simulink model "macroRobot_simulator"  (R2025a)
settings: Solver=FixedStepAuto  StartTime=0.0  StopTime=120  FixedStep=TsControl  MaxStep=0.00025  RelTol=1e-3
PreLoadFcn:
  | initMacroRobotSimulator;
InitFcn:
  | initMacroRobotSimulator;
values from neighbouring files (symbols this model uses):
  initState = deg2rad([-109; +67; +71; -111; -59; +20; -18])    [initMacroRobotSimulator.m]
undefined symbols (not defined in the file or in its folder): smiData, T_b_LaserGate, T_F1_Center, T_F1_Square1, T_F1_Square2, T_F1_Z1, T_F1_Z2, TsControl, X, Y, Z
libraries: sm_lib x50, nesl_utility x13, simulink x1, matrix_library x1, lib_lowLevelController x1, lib_ForwardKinematicsMacroRobot x1, lib_highLevelController x1, lib_InverseKinematicsMacroRobotVelocity x1, lib_saturateMacroRobotPosition x1
(part 1 of 2)
settings Model: Creator=muralikarnam  LastModifiedBy=gordi
settings SolverCC: InitialStep=0.00025  AlgebraicLoopSolver=TrustRegion
settings DataIOCC: ReturnWorkspaceOutputs=off
settings DebuggingCC: UnconnectedInputMsg=warning  UnconnectedOutputMsg=warning  UnconnectedLineMsg=warning  ArithmeticOperatorsInVariantConditions=warning
settings ModelReferenceCC: EnableRefExpFcnMdlSchedulingChecks=on
settings SFSimCC: SimUseLocalCustomCode=off  CustomCodeUndefinedFunction=UseInterfaceOnly
settings RTWCC: RTWUseLocalCustomCode=off  GPUComputeCapability=3.5
settings ExplorerConfigSet: InternalSimMechanicsExplorerSettings="<ExplorerConfiguration><canonicalview>default</canonicalview><AnimationSetting><BasePlaybackSpeed>1.0</BasePlaybackSpeed><PlaybackSpeedFactor>1.0</PlaybackSpeedFactor></AnimationSetting><TilePanel><TileInfo><Tiles Columns=\"2\" Count=\"4\" Rows=\"2\"><Column Weight=\"0.5\"/><Column Weight=\"0.5\"/><Row Weight=\"0.4989\"/><Row Weight=\"0.5011\"/><Tile Height=\"1\" Width=\"1\" X=\"0\" Y=\"0\"/><Tile Height=\"1\" Width=\"1\" X=\"0\" Y=\"1\"/><Tile Height=\"1\" Width=\"1\" X=\"1\" Y=\"0\"/><Tile Height=\"1\" Width=\"1\" X=\"1\" Y=\"1\"/></Tiles></TileInfo><SceneInfo><SceneViewer><BGColor><R>1</R><G>1</G><B>1</B></BGColor><Camera><DoPerspective>off</DoPerspective><Position><X>0.889681490965632871</X><Y>-0.204858956191177222</Y><Z>0.717499386736355049</Z></Position><Center><X>0.12826853071869837</X><Y>0.556554004055757279</Y><Z>-0.0439135735105794234</Z></Center><Up><X>-0.408248290463863073</X><Y>0.408248290463863073</Y><Z>0.816496580927726145</Z></Up><ViewLimDist>1</ViewLimDist><YLim>0.942103152871131888</YLim><XLim>2.08143163867977155</XLim></Camera></SceneViewer><SceneViewer><BGColor><R>1</R><G>1</G><B>1</B></BGColor><Camera><DoPerspective>off</DoPerspective><Position><X>-0.00698647458212509065</X><Y>0.230017892417154979</Y><Z>4.04703777738695258</Z></Position><Center><X>-0.00698647458212509065</X><Y>0.230017892417154979</Y><Z>2.40693099358119156</Z></Center><Up><X>0</X><Y>1</Y><Z>-0</Z></Up><ViewLimDist>1</ViewLimDist><YLim>1.03411994695663445</YLim><XLim>2.27198843364821945</XLim></Camera></SceneViewer><SceneViewer><BGColor><R>1</R><G>1</G><B>1</B></BGColor><Camera><DoPerspective>off</DoPerspective><Position><X>0.153841985146384364</X><Y>-0.651273483880472792</Y><Z>0.065143133491425087</Z></Position><Center><X>0.153841985146384364</X><Y>0.649055207581570759</Y><Z>0.065143133491425087</Z></Center><Up><X>0</X><Y>-0</Y><Z>1</Z></Up><ViewLimDist>1</ViewLimDist><YLim>0.788860071897506732</YLim><XLim>1.74286468221093993</XLim></Camera></SceneViewer><SceneViewer><BGColor><R>1</R><G>1</G><B>1</B></BGColor><Camera><DoPerspective>off</DoPerspective><Position><X>1.46260866869952211</X><Y>0.649055169227639173</Y><Z>0.0651431279093408477</Z></Position><Center><X>0.153841982815738465</X><Y>0.649055169227639173</Y><Z>0.0651431279093408477</Z></Center><Up><X>-0</X><Y>0</Y><Z>1</Z></Up><ViewLimDist>1</ViewLimDist><YLim>0.788860071897506732</YLim><XLim>1.73314610591608353</XLim></Camera></SceneViewer></SceneInfo></TilePanel><MechEditorPanel><Cameras/><GfxPanelCameraMap/><VideoCreator><PlaybackSpeedRatio>1.0</PlaybackSpeedRatio><FrameRate>30</FrameRate><VideoFormat>Motion JPEG AVI</VideoFormat><FrameSize>auto</FrameSize></VideoCreator></MechEditorPanel></ExplorerConfiguration>"

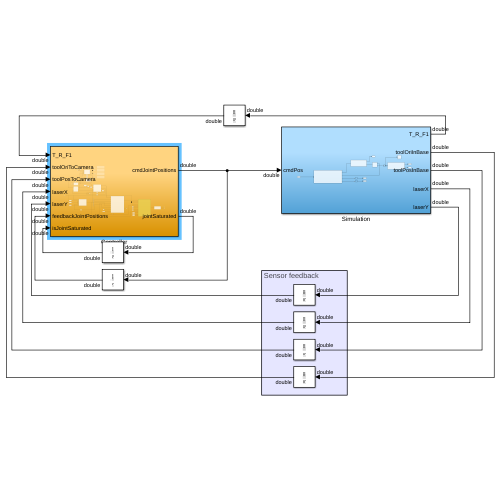
[thumbnail: Simulink's stored preview of the top-level diagram]
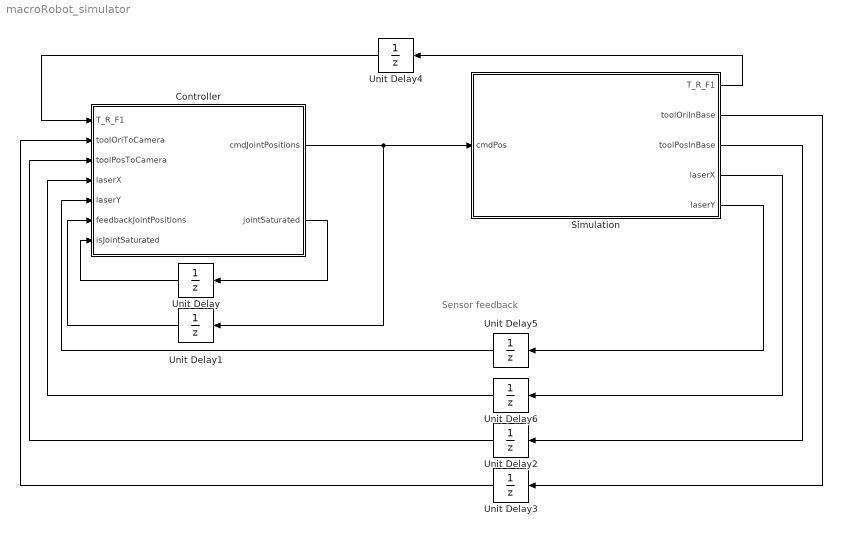
== system macroRobot_simulator ==
  note: Sensor feedback
  Controller : Subsystem
  Simulation : Subsystem
  Unit Delay : UnitDelay  SampleTime=-1  HasFrameUpgradeWarning=on
  Unit Delay1 : UnitDelay  InitialCondition=initState  SampleTime=-1  HasFrameUpgradeWarning=on
  Unit Delay{2..6} (5 alike) : UnitDelay  SampleTime=3 * TsControl  HasFrameUpgradeWarning=on
  wires:
  Controller/1(cmdJointPositions) -> Simulation/1(cmdPos), Unit Delay1/1
  Controller/2(jointSaturated) -> Unit Delay/1
  Unit Delay/1 -> Controller/7(isJointSaturated)
  Unit Delay1/1 -> Controller/6(feedbackJointPositions)
  Simulation/3(toolPosInBase) -> Unit Delay2/1
  Simulation/2(toolOriInBase) -> Unit Delay3/1
  Unit Delay2/1 -> Controller/3(toolPosToCamera)
  Unit Delay3/1 -> Controller/2(toolOriToCamera)
  Simulation/1(T_R_F1) -> Unit Delay4/1
  Unit Delay4/1 -> Controller/1(T_R_F1)
  Simulation/4(laserX) -> Unit Delay6/1
  Simulation/5(laserY) -> Unit Delay5/1
  Unit Delay6/1 -> Controller/4(laserX)
  Unit Delay5/1 -> Controller/5(laserY)

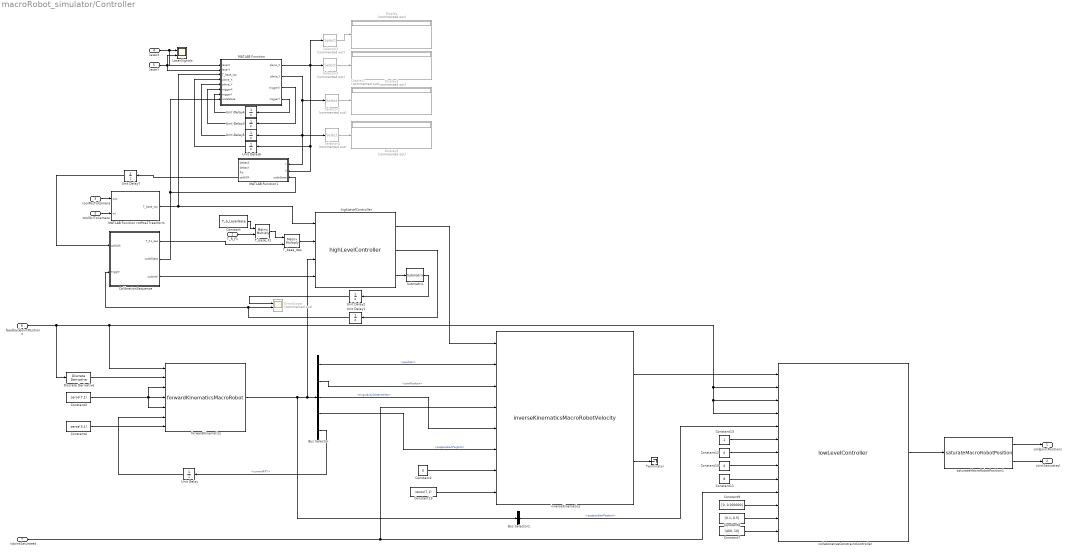
== system macroRobot_simulator/Controller ==
  T_R_F1 : Inport
  toolOriToCamera : Inport  Port=2
  toolPosToCamera : Inport  Port=3
  laserX : Inport  Port=4
  laserY : Inport  Port=5
  feedbackJointPositions : Inport  Port=6
  isJointSaturated : Inport  Port=7
  Bus Selector : BusSelector  OutputSignals=jacobian,jointPosition,singularityDistanceVec,posJacobianPerJoint,currentRPY
  Bus Selector1 : BusSelector  OutputSignals=posJacobianPerJoint
  CalibrationSequence : Stateflow chart  TreatAsAtomicUnit=on
      settings: PortSchema="{\"entries\":[{\"content\":{\"sides\":[{\"content\":{\"connectorIds\":[\"In2\",\"In1\"]},\"type\":\"ConnectorPlacement.EquallySpacedRectSide\",\"uuid\":\"ba4e8509-f946-41ef-8a94-f9774c0ab56e\"},{\"content\":{\"connectorIds\":[\"Out1\",\"Out3\",\"Out2\"],\"side\":\"RIGHT\"},\"type\":\"ConnectorPlacement.EquallySpacedRectSide\",\"uuid\":\"fc30842f-df1e-47fb-bf57-f6f1ca01699a\"},{\"content\":{\"side\":\"TOP\"},\"type\":\"ConnectorPlacement.EquallySpacedRectSide\",\"uuid\":\"47ae690f-5295-4d29-a2fc-2dde971158dc\"}]},\"type\":\"ConnectorPlacement.EquallySpacedConnector\",\"uuid\":\"3427ad9d-5ce5-4e5d-b7e5-c1727f5cb037\"}],\"packageUris\":[\"http://schema.mathworks.com/mf0/Connector/R2020b\"],\"version\":\"1.0\"}"
  Constant : Constant  Value=T_b_LaserGate
  Constant10 : Constant  Value=0  OutDataTypeStr=boolean
  Constant11 : Constant  Value=8  OutDataTypeStr=uint8
  Constant12 : Constant  Value=0  OutDataTypeStr=boolean
  Constant13 : Constant
  Constant15 : Constant  Value=zeros(7,1)
  Constant2 : Constant  Value=0
  Constant3 : Constant  Value=zeros(7,1)
  Constant4 : Constant  Value=zeros(3,1)
  Constant7 : Constant  Value=[400; 10]
  Constant8 : Constant  Value=[0.1; 0.5]
  Constant9 : Constant  Value=[0, 0.000000]
  Discrete Derivative : simulink/Discrete/Discrete Derivative  gainval=1.0  ICPrevScaledInput=0.0  OutMin=[]  OutMax=[]  OutDataType=fixdt(1, 16)  OutScaling=2^-10  DoSatur=off
  Display{,1..3} (4 alike) : Display  Commented=on
  ErrorScope : Scope  Commented=on  NumInputPorts=2
      settings: Title=ErrorPose & trigger  ActiveDisplayYMinimum=-1.2794998753501146  ActiveDisplayYMaximum=2.7547759189623635
  LaserSignals : Scope  NumInputPorts=2
      settings: Title=ErrorPose & trigger  ActiveDisplayYMinimum=-1.1952916064245291  ActiveDisplayYMaximum=2.3134323945660178  DataLoggingVariableName=ScopeData2
  MATLAB Function : MATLAB Function  TreatAsAtomicUnit=on
  MATLAB Function rotPos2Trasnform : MATLAB Function  TreatAsAtomicUnit=on
  MATLAB Function1 : MATLAB Function  TreatAsAtomicUnit=on
  Selector1 : Selector  Commented=on  NumberOfDimensions=3  InputPortWidth=3  IndexOptions=Index vector (dialog),Index vector (dialog),Index vector (dialog)  Indices=[1 2 3],[1 2],1  OutputSizes=1,1,1
  Selector2 : Selector  Commented=on  NumberOfDimensions=3  InputPortWidth=3  IndexOptions=Index vector (dialog),Index vector (dialog),Index vector (dialog)  Indices=[1 2 3],[1 2],1  OutputSizes=1,1,1
  Selector3 : Selector  Commented=on  NumberOfDimensions=3  InputPortWidth=3  IndexOptions=Index vector (dialog),Index vector (dialog),Index vector (dialog)  Indices=[1 2 3],[1 2],2  OutputSizes=1,1,1
  Selector4 : Selector  Commented=on  NumberOfDimensions=3  InputPortWidth=3  IndexOptions=Index vector (dialog),Index vector (dialog),Index vector (dialog)  Indices=[1 2 3],[1 2],2  OutputSizes=1,1,1
  Submatrix : matrix_library/Submatrix  RowSpan=Range of rows  RowStartMode=First  RowStartIndex=1  RowEndMode=Index  RowEndIndex=3  ColSpan=All columns  ColStartMode=First  ColStartIndex=1  ColEndMode=Last  ColEndIndex=1
  T_base_F1 : Product  Multiplication=Matrix(*)
  T_base_des : Product  Multiplication=Matrix(*)
  Terminator : Terminator
  Unit Delay{,1..4,7} (6 alike) : UnitDelay  SampleTime=-1  HasFrameUpgradeWarning=on
  Unit Delay5 : UnitDelay  InitialCondition=zeros(3,2,2,3)  SampleTime=-1  HasFrameUpgradeWarning=on
  Unit Delay6 : UnitDelay  InitialCondition=zeros(3,2,2,3)  SampleTime=-1  HasFrameUpgradeWarning=on
  collaborativeConstraintController : lib_lowLevelController/lowLevelController  SystemSampleTime=-1  VariantActivationTime=update diagram  EmptyChoice=off  PassThrough=off  PassThroughVariantControl=(default)  EmptyChoiceVariantControl=(default)  AllowFlexibleInterface=on  Latency=0  AutoFrameSizeCalculation=off
  forwardKinematics : lib_ForwardKinematicsMacroRobot/forwardKinematicsMacroRobot  SystemSampleTime=-1  VariantActivationTime=update diagram  EmptyChoice=off  PassThrough=off  PassThroughVariantControl=(default)  EmptyChoiceVariantControl=(default)  AllowFlexibleInterface=on  Latency=0  AutoFrameSizeCalculation=off
  highLevelController : lib_highLevelController/highLevelController  SystemSampleTime=-1  VariantActivationTime=update diagram  EmptyChoice=off  PassThrough=off  PassThroughVariantControl=(default)  EmptyChoiceVariantControl=(default)  AllowFlexibleInterface=on  Latency=0  AutoFrameSizeCalculation=off
  inverseKinematics : lib_InverseKinematicsMacroRobotVelocity/inverseKinematicsMacroRobotVelocity  SystemSampleTime=-1  VariantActivationTime=update diagram  EmptyChoice=off  PassThrough=off  PassThroughVariantControl=(default)  EmptyChoiceVariantControl=(default)  AllowFlexibleInterface=on  Latency=0  AutoFrameSizeCalculation=off
  saturateMacroRobotPosition1 : lib_saturateMacroRobotPosition/saturateMacroRobotPosition  SystemSampleTime=-1  VariantActivationTime=update diagram  EmptyChoice=off  PassThrough=off  PassThroughVariantControl=(default)  EmptyChoiceVariantControl=(default)  AllowFlexibleInterface=on  Latency=0  AutoFrameSizeCalculation=off
  cmdJointPositions : Outport  VectorParamsAs1DForOutWhenUnconnected=off
  jointSaturated : Outport  Port=2  VectorParamsAs1DForOutWhenUnconnected=off
  wires:
  feedbackJointPositions/1 -> Discrete Derivative/1, collaborativeConstraintController/2, collaborativeConstraintController/3, collaborativeConstraintController/4, forwardKinematics/1
  Unit Delay/1 -> forwardKinematics/6
  Bus Selector/1 -> inverseKinematics/2  "<jacobian>"
  Constant8/1 -> collaborativeConstraintController/12
  Constant2/1 -> inverseKinematics/7
  inverseKinematics/1 -> collaborativeConstraintController/1
  Constant7/1 -> collaborativeConstraintController/13
  Constant3/1 -> forwardKinematics/3, forwardKinematics/5, forwardKinematics/4
  Bus Selector/2 -> inverseKinematics/3  "<jointPosition>"
  Bus Selector/5 -> Unit Delay/1  "<currentRPY>"
  Constant9/1 -> collaborativeConstraintController/11
  Discrete Derivative/1 -> forwardKinematics/2
  Constant12/1 -> collaborativeConstraintController/7
  Constant4/1 -> forwardKinematics/7
  forwardKinematics/1 -> highLevelController/3, Bus Selector/1, Bus Selector1/1
  Constant11/1 -> collaborativeConstraintController/9
  Constant10/1 -> collaborativeConstraintController/8
  Constant13/1 -> collaborativeConstraintController/6
  Bus Selector1/1 -> collaborativeConstraintController/5  "<posJacobianPerJoint>"
  Bus Selector/4 -> inverseKinematics/6  "<posJacobianPerJoint>"
  inverseKinematics/2 -> Terminator/1
  Bus Selector/3 -> inverseKinematics/5  "<singularityDistanceVec>"
  isJointSaturated/1 -> inverseKinematics/4, collaborativeConstraintController/10
  Constant15/1 -> inverseKinematics/8
  saturateMacroRobotPosition1/1 -> cmdJointPositions/1
  collaborativeConstraintController/1 -> saturateMacroRobotPosition1/1
  saturateMacroRobotPosition1/2 -> jointSaturated/1
  highLevelController/1 -> inverseKinematics/1
  toolOriToCamera/1 -> MATLAB Function rotPos2Trasnform/2(ori)
  toolPosToCamera/1 -> MATLAB Function rotPos2Trasnform/1(pos)
  MATLAB Function rotPos2Trasnform/1(T_base_tcp) -> highLevelController/1, MATLAB Function/3(T_base_tcp)
  highLevelController/2 -> Unit Delay1/1
  Unit Delay1/1 -> CalibrationSequence/1(trigger), ErrorScope/2
  Constant/1 -> T_base_F1/1
  T_base_F1/1 -> T_base_des/1
  T_R_F1/1 -> T_base_F1/2
  T_base_des/1 -> highLevelController/2
  CalibrationSequence/1(T_F1_des) -> T_base_des/2
  highLevelController/3 -> Submatrix/1
  Unit Delay2/1 -> ErrorScope/1
  Submatrix/1 -> Unit Delay2/1
  CalibrationSequence/2(codeVel) -> highLevelController/4
  laserY/1 -> MATLAB Function/2(laserY), LaserSignals/2
  laserX/1 -> MATLAB Function/1(laserX), LaserSignals/1
  MATLAB Function/4(triggerY) -> Unit Delay4/1
  Unit Delay3/1 -> MATLAB Function/6("triggerX ")
  Unit Delay4/1 -> MATLAB Function/7("triggerY ")
  MATLAB Function/1(plane_X) -> Selector2/1, Selector3/1, MATLAB Function1/2(X), Unit Delay6/1
  MATLAB Function/2(plane_Y) -> MATLAB Function1/1(Y), Unit Delay5/1, Selector4/1, Selector1/1
  MATLAB Function/3(triggerX) -> Unit Delay3/1
  Selector2/1 -> Display/1
  Selector1/1 -> Display1/1
  CalibrationSequence/3(codeState) -> MATLAB Function/8(codeState), MATLAB Function1/3(codeState)
  Selector3/1 -> Display2/1
  Selector4/1 -> Display3/1
  Unit Delay5/1 -> MATLAB Function/5("plane_Y ")
  Unit Delay6/1 -> MATLAB Function/4("plane_X ")
  MATLAB Function1/4(calibOK) -> Unit Delay7/1
  Unit Delay7/1 -> CalibrationSequence/2(calibOK)

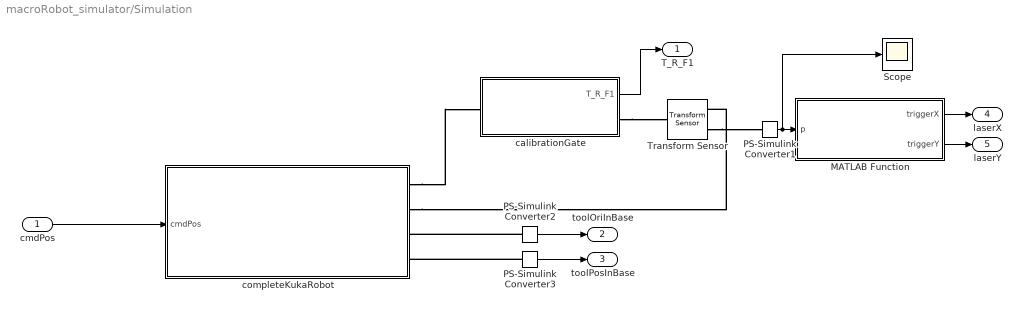
== system macroRobot_simulator/Simulation ==
  cmdPos : Inport
  MATLAB Function : MATLAB Function  TreatAsAtomicUnit=on
  PS-Simulink Converter1 : nesl_utility/PS-Simulink Converter  PhysicalDomain=network_engine_domain  SubClassName=ps_output  LeftPortType=input  RightPortType=output  PseudoPeriodic=off  Frequencies=[]  VectorFormat=inherit  Unit=inherit  AffineConversion=off
  PS-Simulink Converter2 : nesl_utility/PS-Simulink Converter  PhysicalDomain=network_engine_domain  SubClassName=ps_output  LeftPortType=input  RightPortType=output  PseudoPeriodic=off  Frequencies=[]  VectorFormat=inherit  Unit=inherit  AffineConversion=off
  PS-Simulink Converter3 : nesl_utility/PS-Simulink Converter  PhysicalDomain=network_engine_domain  SubClassName=ps_output  LeftPortType=input  RightPortType=output  PseudoPeriodic=off  Frequencies=[]  VectorFormat=inherit  Unit=inherit  AffineConversion=off
  Scope : Scope
  Transform Sensor : sm_lib/Frames and Transforms/Transform Sensor  MeasurementFrame=World  RotationSequence=XYX  SenseAngle=off  SenseAxis=off  SenseQ=off  SenseR=off  SenseRotationSequence=off  SenseOmegaX=off  SenseOmegaY=off  SenseOmegaZ=off  SenseOmega=off  SenseQDot=off  SenseRDot=off  SenseRotationSequenceDot=off  SenseAlphaX=off  SenseAlphaY=off  SenseAlphaZ=off  SenseAlpha=off  SenseQDDot=off  SenseRDDot=off  SenseX=off  SenseY=off  SenseZ=off  SenseXYZ=on  SenseRad=off  SenseAzim=off  SenseDist=off  SenseInc=off  SenseXDot=off  SenseYDot=off  SenseZDot=off  SenseXYZDot=off  SenseRadDot=off  SenseAzimDot=off  SenseDistDot=off  SenseIncDot=off  SenseXDDot=off  SenseYDDot=off  SenseZDDot=off  SenseXYZDDot=off  SenseRadDDot=off  SenseAzimDDot=off  SenseDistDDot=off  SenseIncDDot=off
  calibrationGate : Subsystem
  completeKukaRobot : Subsystem
  T_R_F1 : Outport
  toolOriInBase : Outport  Port=2
  toolPosInBase : Outport  Port=3
  laserX : Outport  Port=4
  laserY : Outport  Port=5
  wires:
  cmdPos/1 -> completeKukaRobot/1(cmdPos)
  PS-Simulink Converter3/1 -> toolPosInBase/1
  PS-Simulink Converter2/1 -> toolOriInBase/1
  calibrationGate/1(T_R_F1) -> T_R_F1/1
  PS-Simulink Converter1/1 -> Scope/1, MATLAB Function/1(p)
  MATLAB Function/1(triggerX) -> laserX/1
  MATLAB Function/2(triggerY) -> laserY/1
  connections:
  PS-Simulink Converter3/LConn1 -- completeKukaRobot/RConn4
  PS-Simulink Converter2/LConn1 -- completeKukaRobot/RConn3
  completeKukaRobot/RConn1 -- calibrationGate/LConn1
  completeKukaRobot/RConn2 -- Transform Sensor/RConn1
  calibrationGate/RConn1 -- Transform Sensor/LConn1
  Transform Sensor/RConn2 -- PS-Simulink Converter1/LConn1

== system macroRobot_simulator/Simulation/calibrationGate ==
  laserGate : Subsystem
  tableFrame : PMIOPort  Side=Left
  LaserGate_F1 : PMIOPort  Port=2  Side=Right
  T_R_F1 : Outport
  wires:
  laserGate/1(T_R_F1) -> T_R_F1/1
  connections:
  laserGate/LConn1 -- tableFrame/RConn1
  LaserGate_F1/RConn1 -- laserGate/RConn1

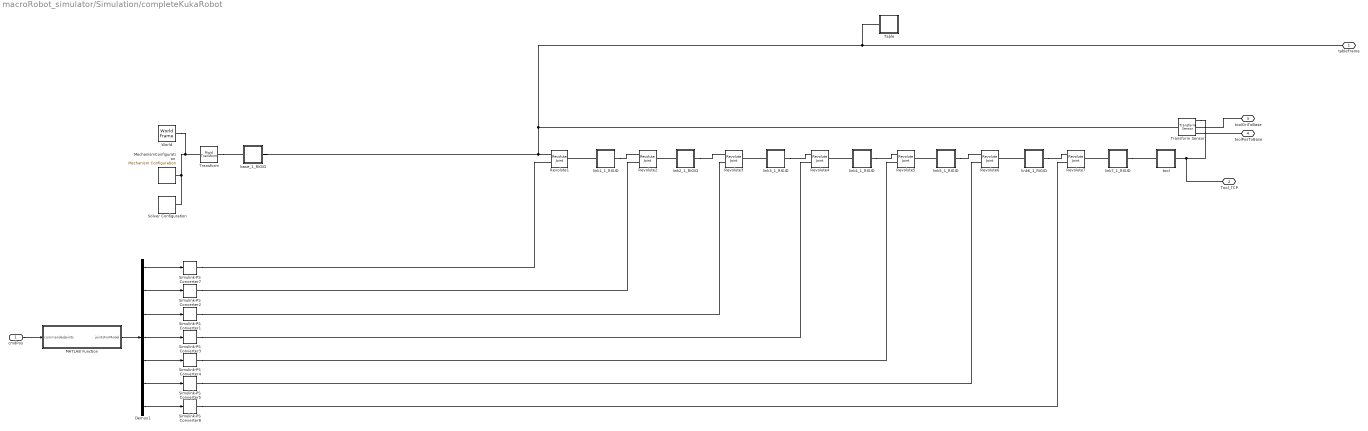
== system macroRobot_simulator/Simulation/completeKukaRobot ==
  cmdPos : Inport  PortDimensions=[7 1]
  Demux1 : Demux  Outputs=7
  MATLAB Function : MATLAB Function  TreatAsAtomicUnit=on
  MechanismConfiguration : sm_lib/Utilities/Mechanism Configuration  UniformGravity=Constant  GravityVector=[0 -9.80665 0]  GravityVectorUnits=m/s^2  LinearizationDelta=0.001  JointModeTransitionNonlinearIterations=2
  Revolute1 : sm_lib/Joints/Revolute Joint  JointMode=Normal  CompositeWrenchDir=FollowerOnBase  CompositeWrenchFrame=BaseFrame  SenseConstraintForce=off  SenseConstraintTorque=off  SenseTotalForce=off  SenseTotalTorque=off  PositionTargetSpecify=on  PositionTargetPriority=Low  PositionTargetValue=initState(1)  PositionTargetValueUnits=rad  VelocityTargetSpecify=off  VelocityTargetPriority=High  VelocityTargetValue=0  VelocityTargetValueUnits=deg/s  EquilibriumPosition=0  EquilibriumPositionUnits=rad  SpringStiffness=0  SpringStiffnessUnits=N*m/rad  DampingCoefficient=0  DampingCoefficientUnits=N*m/(rad/s)  LowerLimitSpecify=off  LowerLimitBound=-90  LowerLimitBoundUnits=deg  LowerLimitStiffness=1e4  LowerLimitStiffnessUnits=N*m/deg  LowerLimitDamping=10  LowerLimitDampingUnits=N*m/(deg/s)  LowerLimitTransitionRegionWidth=0.1  LowerLimitTransitionRegionWidthUnits=deg  UpperLimitSpecify=off  UpperLimitBound=90  UpperLimitBoundUnits=deg  UpperLimitStiffness=1e4  UpperLimitStiffnessUnits=N*m/deg  UpperLimitDamping=10  UpperLimitDampingUnits=N*m/(deg/s)  UpperLimitTransitionRegionWidth=0.1  UpperLimitTransitionRegionWidthUnits=deg  TorqueActuationMode=ComputedTorque  MotionActuationMode=InputMotion  SensePosition=off  SenseVelocity=off  SenseAcceleration=off  SenseTorqueForce=off  SenseLowerLimitTorqueForce=off  SenseUpperLimitTorqueForce=off
  Revolute2 : sm_lib/Joints/Revolute Joint  JointMode=Normal  CompositeWrenchDir=FollowerOnBase  CompositeWrenchFrame=BaseFrame  SenseConstraintForce=off  SenseConstraintTorque=off  SenseTotalForce=off  SenseTotalTorque=off  PositionTargetSpecify=on  PositionTargetPriority=Low  PositionTargetValue=initState(2)  PositionTargetValueUnits=rad  VelocityTargetSpecify=off  VelocityTargetPriority=High  VelocityTargetValue=0  VelocityTargetValueUnits=deg/s  EquilibriumPosition=0  EquilibriumPositionUnits=rad  SpringStiffness=0  SpringStiffnessUnits=N*m/rad  DampingCoefficient=0  DampingCoefficientUnits=N*m/(rad/s)  LowerLimitSpecify=off  LowerLimitBound=-90  LowerLimitBoundUnits=deg  LowerLimitStiffness=1e4  LowerLimitStiffnessUnits=N*m/deg  LowerLimitDamping=10  LowerLimitDampingUnits=N*m/(deg/s)  LowerLimitTransitionRegionWidth=0.1  LowerLimitTransitionRegionWidthUnits=deg  UpperLimitSpecify=off  UpperLimitBound=90  UpperLimitBoundUnits=deg  UpperLimitStiffness=1e4  UpperLimitStiffnessUnits=N*m/deg  UpperLimitDamping=10  UpperLimitDampingUnits=N*m/(deg/s)  UpperLimitTransitionRegionWidth=0.1  UpperLimitTransitionRegionWidthUnits=deg  TorqueActuationMode=ComputedTorque  MotionActuationMode=InputMotion  SensePosition=off  SenseVelocity=off  SenseAcceleration=off  SenseTorqueForce=off  SenseLowerLimitTorqueForce=off  SenseUpperLimitTorqueForce=off
  Revolute3 : sm_lib/Joints/Revolute Joint  JointMode=Normal  CompositeWrenchDir=FollowerOnBase  CompositeWrenchFrame=BaseFrame  SenseConstraintForce=off  SenseConstraintTorque=off  SenseTotalForce=off  SenseTotalTorque=off  PositionTargetSpecify=on  PositionTargetPriority=Low  PositionTargetValue=initState(3)  PositionTargetValueUnits=rad  VelocityTargetSpecify=off  VelocityTargetPriority=High  VelocityTargetValue=0  VelocityTargetValueUnits=deg/s  EquilibriumPosition=0  EquilibriumPositionUnits=rad  SpringStiffness=0  SpringStiffnessUnits=N*m/rad  DampingCoefficient=0  DampingCoefficientUnits=N*m/(rad/s)  LowerLimitSpecify=off  LowerLimitBound=-90  LowerLimitBoundUnits=deg  LowerLimitStiffness=1e4  LowerLimitStiffnessUnits=N*m/deg  LowerLimitDamping=10  LowerLimitDampingUnits=N*m/(deg/s)  LowerLimitTransitionRegionWidth=0.1  LowerLimitTransitionRegionWidthUnits=deg  UpperLimitSpecify=off  UpperLimitBound=90  UpperLimitBoundUnits=deg  UpperLimitStiffness=1e4  UpperLimitStiffnessUnits=N*m/deg  UpperLimitDamping=10  UpperLimitDampingUnits=N*m/(deg/s)  UpperLimitTransitionRegionWidth=0.1  UpperLimitTransitionRegionWidthUnits=deg  TorqueActuationMode=ComputedTorque  MotionActuationMode=InputMotion  SensePosition=off  SenseVelocity=off  SenseAcceleration=off  SenseTorqueForce=off  SenseLowerLimitTorqueForce=off  SenseUpperLimitTorqueForce=off
  Revolute4 : sm_lib/Joints/Revolute Joint  JointMode=Normal  CompositeWrenchDir=FollowerOnBase  CompositeWrenchFrame=BaseFrame  SenseConstraintForce=off  SenseConstraintTorque=off  SenseTotalForce=off  SenseTotalTorque=off  PositionTargetSpecify=on  PositionTargetPriority=Low  PositionTargetValue=-initState(4)  PositionTargetValueUnits=rad  VelocityTargetSpecify=off  VelocityTargetPriority=High  VelocityTargetValue=0  VelocityTargetValueUnits=deg/s  EquilibriumPosition=0  EquilibriumPositionUnits=rad  SpringStiffness=0  SpringStiffnessUnits=N*m/rad  DampingCoefficient=0  DampingCoefficientUnits=N*m/(rad/s)  LowerLimitSpecify=off  LowerLimitBound=-90  LowerLimitBoundUnits=deg  LowerLimitStiffness=1e4  LowerLimitStiffnessUnits=N*m/deg  LowerLimitDamping=10  LowerLimitDampingUnits=N*m/(deg/s)  LowerLimitTransitionRegionWidth=0.1  LowerLimitTransitionRegionWidthUnits=deg  UpperLimitSpecify=off  UpperLimitBound=90  UpperLimitBoundUnits=deg  UpperLimitStiffness=1e4  UpperLimitStiffnessUnits=N*m/deg  UpperLimitDamping=10  UpperLimitDampingUnits=N*m/(deg/s)  UpperLimitTransitionRegionWidth=0.1  UpperLimitTransitionRegionWidthUnits=deg  TorqueActuationMode=ComputedTorque  MotionActuationMode=InputMotion  SensePosition=off  SenseVelocity=off  SenseAcceleration=off  SenseTorqueForce=off  SenseLowerLimitTorqueForce=off  SenseUpperLimitTorqueForce=off
  Revolute5 : sm_lib/Joints/Revolute Joint  JointMode=Normal  CompositeWrenchDir=FollowerOnBase  CompositeWrenchFrame=BaseFrame  SenseConstraintForce=off  SenseConstraintTorque=off  SenseTotalForce=off  SenseTotalTorque=off  PositionTargetSpecify=on  PositionTargetPriority=Low  PositionTargetValue=initState(5)  PositionTargetValueUnits=rad  VelocityTargetSpecify=off  VelocityTargetPriority=High  VelocityTargetValue=0  VelocityTargetValueUnits=deg/s  EquilibriumPosition=0  EquilibriumPositionUnits=rad  SpringStiffness=0  SpringStiffnessUnits=N*m/rad  DampingCoefficient=0  DampingCoefficientUnits=N*m/(rad/s)  LowerLimitSpecify=off  LowerLimitBound=-90  LowerLimitBoundUnits=deg  LowerLimitStiffness=1e4  LowerLimitStiffnessUnits=N*m/deg  LowerLimitDamping=10  LowerLimitDampingUnits=N*m/(deg/s)  LowerLimitTransitionRegionWidth=0.1  LowerLimitTransitionRegionWidthUnits=deg  UpperLimitSpecify=off  UpperLimitBound=90  UpperLimitBoundUnits=deg  UpperLimitStiffness=1e4  UpperLimitStiffnessUnits=N*m/deg  UpperLimitDamping=10  UpperLimitDampingUnits=N*m/(deg/s)  UpperLimitTransitionRegionWidth=0.1  UpperLimitTransitionRegionWidthUnits=deg  TorqueActuationMode=ComputedTorque  MotionActuationMode=InputMotion  SensePosition=off  SenseVelocity=off  SenseAcceleration=off  SenseTorqueForce=off  SenseLowerLimitTorqueForce=off  SenseUpperLimitTorqueForce=off
  Revolute6 : sm_lib/Joints/Revolute Joint  JointMode=Normal  CompositeWrenchDir=FollowerOnBase  CompositeWrenchFrame=BaseFrame  SenseConstraintForce=off  SenseConstraintTorque=off  SenseTotalForce=off  SenseTotalTorque=off  PositionTargetSpecify=on  PositionTargetPriority=Low  PositionTargetValue=initState(6)  PositionTargetValueUnits=rad  VelocityTargetSpecify=off  VelocityTargetPriority=High  VelocityTargetValue=0  VelocityTargetValueUnits=deg/s  EquilibriumPosition=0  EquilibriumPositionUnits=rad  SpringStiffness=0  SpringStiffnessUnits=N*m/rad  DampingCoefficient=0  DampingCoefficientUnits=N*m/(rad/s)  LowerLimitSpecify=off  LowerLimitBound=-90  LowerLimitBoundUnits=deg  LowerLimitStiffness=1e4  LowerLimitStiffnessUnits=N*m/deg  LowerLimitDamping=10  LowerLimitDampingUnits=N*m/(deg/s)  LowerLimitTransitionRegionWidth=0.1  LowerLimitTransitionRegionWidthUnits=deg  UpperLimitSpecify=off  UpperLimitBound=90  UpperLimitBoundUnits=deg  UpperLimitStiffness=1e4  UpperLimitStiffnessUnits=N*m/deg  UpperLimitDamping=10  UpperLimitDampingUnits=N*m/(deg/s)  UpperLimitTransitionRegionWidth=0.1  UpperLimitTransitionRegionWidthUnits=deg  TorqueActuationMode=ComputedTorque  MotionActuationMode=InputMotion  SensePosition=off  SenseVelocity=off  SenseAcceleration=off  SenseTorqueForce=off  SenseLowerLimitTorqueForce=off  SenseUpperLimitTorqueForce=off
  Revolute7 : sm_lib/Joints/Revolute Joint  JointMode=Normal  CompositeWrenchDir=FollowerOnBase  CompositeWrenchFrame=BaseFrame  SenseConstraintForce=off  SenseConstraintTorque=off  SenseTotalForce=off  SenseTotalTorque=off  PositionTargetSpecify=on  PositionTargetPriority=Low  PositionTargetValue=initState(7)  PositionTargetValueUnits=rad  VelocityTargetSpecify=off  VelocityTargetPriority=High  VelocityTargetValue=0  VelocityTargetValueUnits=deg/s  EquilibriumPosition=0  EquilibriumPositionUnits=rad  SpringStiffness=0  SpringStiffnessUnits=N*m/rad  DampingCoefficient=0  DampingCoefficientUnits=N*m/(rad/s)  LowerLimitSpecify=off  LowerLimitBound=-90  LowerLimitBoundUnits=deg  LowerLimitStiffness=1e4  LowerLimitStiffnessUnits=N*m/deg  LowerLimitDamping=10  LowerLimitDampingUnits=N*m/(deg/s)  LowerLimitTransitionRegionWidth=0.1  LowerLimitTransitionRegionWidthUnits=deg  UpperLimitSpecify=off  UpperLimitBound=90  UpperLimitBoundUnits=deg  UpperLimitStiffness=1e4  UpperLimitStiffnessUnits=N*m/deg  UpperLimitDamping=10  UpperLimitDampingUnits=N*m/(deg/s)  UpperLimitTransitionRegionWidth=0.1  UpperLimitTransitionRegionWidthUnits=deg  TorqueActuationMode=ComputedTorque  MotionActuationMode=InputMotion  SensePosition=off  SenseVelocity=off  SenseAcceleration=off  SenseTorqueForce=off  SenseLowerLimitTorqueForce=off  SenseUpperLimitTorqueForce=off
  Simulink-PS Converter{1..5,7..8} (7 alike) : nesl_utility/Simulink-PS Converter  PhysicalDomain=network_engine_domain  SubClassName=ps_input  LeftPortType=input  RightPortType=output  PseudoPeriodic=off  Frequencies=[]  NoiseDistribution=none  NoiseParameters=[]  Unit=1  AffineConversion=off  FilteringAndDerivatives=filter  SimscapeFilterOrder=2  InputFilterTimeConstant=0.001  UdotUserProvided=0
  Solver Configuration : nesl_utility/Solver Configuration  PhysicalDomain=network_engine_domain  SubClassName=solver  LeftPortType=input  RightPortType=generic  Tones=[]  Harmonics=[]  SimulateNoise=off  Profile=off  UseLocalSampling=off  EnableSwitchedLinearOptims=on  FrequencyDomain=off  UseCCode=off  RelTol=0.001  AbsTol=0.001  MinStep=1e-09  ToWorkspace=off  RevertToSquareIcSolve=off  NumHomotopyIterations=100  PhasorMode=off  PhasorModeNumHarmonics=1  ConsistencySolver=NEWTON_XTOL_AFTER_FTOL  IndexReductionMethod=DerivativeReplacement  DoDC=off  ResidualTolerance=1e-09  ConsistencyTolSource=GLOBAL  ConsistencyAbsTol=0.001  ConsistencyRelTol=0.001  ConsistencyTolFactor=0.001  UseLocalSolver=off  LocalSolverChoice=NE_BACKWARD_EULER_ADVANCER  ResolveIndetEquations=on  FunctionEvalNumThread=1  LocalSolverSampleTime=0.001  DoFixedCost=off  MaxNonlinIter=3  MaxModeIter=2  ComputeImpulses=off  ImpulseIterations=2  LinearAlgebra=auto  LinearAlgebraNumThread=0  EquationFormulation=NE_TIME_EF  DelaysMemoryBudget=1024  AutomaticFiltering=on  FilteringTimeConstant=0.001  PartitionStorageMethod=AS_NEEDED  PartitionMemoryBudget=1024  PartitionMethod=ROBUST  MultibodyUseLocalSolver=off  MultibodyLocalSolverChoice=ODE1  MultibodyLocalSolverSampleTime=0.001
  Table : Subsystem
  Transform : sm_lib/Frames and Transforms/Rigid Transform  RotationMethod=ArbitraryAxis  FollAlignAxisA=+X  BaseAlignAxisA=+Y  FollAlignAxisB=+Y  BaseAlignAxisB=+Z  RotationStandardAxis=+Z  RotationAngle=smiData.RigidTransform(15).angle  RotationAngleUnits=rad  RotationArbitraryAxis=smiData.RigidTransform(15).axis  RotationSequenceAxes=FollowerAxes  RotationSequence=XYX  RotationSequenceAngles=[0 0 0]  RotationSequenceAnglesUnits=deg  RotationMatrix=[1 0 0; 0 1 0; 0 0 1]  Quaternion=[1 0 0 0]  TranslationMethod=Cartesian  TranslationCartesianOffset=smiData.RigidTransform(15).translation  TranslationCartesianOffsetUnits=mm  TranslationStandardAxis=+Z  TranslationStandardOffset=0  TranslationStandardOffsetUnits=m  TranslationROffset=0  TranslationROffsetUnits=m  TranslationThetaOffset=0  TranslationThetaOffsetUnits=deg  TranslationZOffset=0  TranslationZOffsetUnits=m
  Transform Sensor : sm_lib/Frames and Transforms/Transform Sensor  MeasurementFrame=Base  RotationSequence=XYX  SenseAngle=off  SenseAxis=off  SenseQ=off  SenseR=on  SenseRotationSequence=off  SenseOmegaX=off  SenseOmegaY=off  SenseOmegaZ=off  SenseOmega=off  SenseQDot=off  SenseRDot=off  SenseRotationSequenceDot=off  SenseAlphaX=off  SenseAlphaY=off  SenseAlphaZ=off  SenseAlpha=off  SenseQDDot=off  SenseRDDot=off  SenseX=off  SenseY=off  SenseZ=off  SenseXYZ=on  SenseRad=off  SenseAzim=off  SenseDist=off  SenseInc=off  SenseXDot=off  SenseYDot=off  SenseZDot=off  SenseXYZDot=off  SenseRadDot=off  SenseAzimDot=off  SenseDistDot=off  SenseIncDot=off  SenseXDDot=off  SenseYDDot=off  SenseZDDot=off  SenseXYZDDot=off  SenseRadDDot=off  SenseAzimDDot=off  SenseDistDDot=off  SenseIncDDot=off
  World : sm_lib/Frames and Transforms/World Frame
  base_1_RIGID : Subsystem
  link1_1_RIGID : Subsystem
  link2_1_RIGID : Subsystem
  link3_1_RIGID : Subsystem
  link4_1_RIGID : Subsystem
  link5_1_RIGID : Subsystem
  link6_1_RIGID : Subsystem
  link7_1_RIGID : Subsystem
  tool : Subsystem
  tableFrame : PMIOPort  Side=Right
  Tool_TCP : PMIOPort  Port=2  Side=Right
  toolOriToBase : PMIOPort  Port=3  Side=Right
  toolPosToBase : PMIOPort  Port=4  Side=Right
  wires:
  cmdPos/1 -> MATLAB Function/1(commandedJoints)
  Demux1/7 -> Simulink-PS Converter8/1
  Demux1/6 -> Simulink-PS Converter5/1
  Demux1/5 -> Simulink-PS Converter4/1
  Demux1/4 -> Simulink-PS Converter3/1
  Demux1/3 -> Simulink-PS Converter1/1
  Demux1/2 -> Simulink-PS Converter2/1
  Demux1/1 -> Simulink-PS Converter7/1
  MATLAB Function/1(jointsForModel) -> Demux1/1
  connections:
  Simulink-PS Converter2/RConn1 -- Revolute2/LConn2
  Simulink-PS Converter3/RConn1 -- Revolute4/LConn2
  Simulink-PS Converter5/RConn1 -- Revolute6/LConn2
  Simulink-PS Converter1/RConn1 -- Revolute3/LConn2
  Simulink-PS Converter4/RConn1 -- Revolute5/LConn2
  Simulink-PS Converter8/RConn1 -- Revolute7/LConn2
  Simulink-PS Converter7/RConn1 -- Revolute1/LConn2
  link5_1_RIGID/LConn1 -- Revolute5/RConn1
  link2_1_RIGID/LConn1 -- Revolute2/RConn1
  link4_1_RIGID/RConn1 -- Revolute5/LConn1
  link1_1_RIGID/RConn1 -- Revolute2/LConn1
  link6_1_RIGID/RConn1 -- Revolute7/LConn1
  link3_1_RIGID/RConn1 -- Revolute4/LConn1
  Transform Sensor/LConn1 -- tableFrame/RConn1 -- Table/LConn1 -- base_1_RIGID/RConn1 -- Revolute1/LConn1
  link1_1_RIGID/LConn1 -- Revolute1/RConn1
  link3_1_RIGID/LConn1 -- Revolute3/RConn1
  link5_1_RIGID/RConn1 -- Revolute6/LConn1
  link7_1_RIGID/LConn1 -- Revolute7/RConn1
  link2_1_RIGID/RConn1 -- Revolute3/LConn1
  link4_1_RIGID/LConn1 -- Revolute4/RConn1
  link6_1_RIGID/LConn1 -- Revolute6/RConn1
  link7_1_RIGID/RConn1 -- tool/LConn1
  Transform Sensor/RConn1 -- Tool_TCP/RConn1 -- tool/RConn1
  toolOriToBase/RConn1 -- Transform Sensor/RConn2
  toolPosToBase/RConn1 -- Transform Sensor/RConn3
  Solver Configuration/RConn1 -- MechanismConfiguration/RConn1 -- World/RConn1 -- Transform/LConn1
  Transform/RConn1 -- base_1_RIGID/LConn1

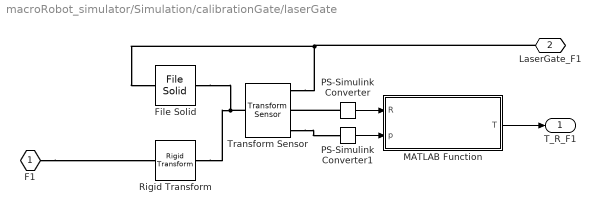
== system macroRobot_simulator/Simulation/calibrationGate/laserGate ==
  File Solid : sm_lib/Body Elements/File Solid  ExtGeomFileName=ORL2-40T-2PS6.STEP  UnitType=FromFile  ExtGeomFileUnits=m  StepReaderType=HEX  ExportConvexHullGeometry=off  InertiaType=PointMass  BasedOnType=DensityFromFile  Density=1000  DensityUnits=kg/m^3  Mass=1  MassUnits=kg  CenterOfMass=[0 0 0]  CenterOfMassUnits=m  MomentsOfInertia=[1 1 1]  MomentsOfInertiaUnits=kg*m^2  ProductsOfInertia=[0 0 0]  ProductsOfInertiaUnits=kg*m^2  GraphicType=FromGeometry  MarkerShape=Sphere  MarkerSize=10  GraphicVisPropType=SimpleVisualProperties  GraphicDiffuseColor=[0.5 0.5 0.5]  GraphicOpacity=1  GraphicSpecularColor=[0.5 0.5 0.5 1.0]  GraphicAmbientColor=[0.15 0.15 0.15 1.0]  GraphicEmissiveColor=[0.0 0.0 0.0 1.0]  GraphicShininess=75  DoExposeReferenceFrame=on  SerializedFrames=<Frames><Frame><Id>Frame1</Id><Value><Name>F1</Name><Origin><Source>ReferenceFrame</Source><FeatureName>circular curve 214</FeatureName></Origin><PrimaryAxis><DefinedDirection>+X</DefinedDirection><Source>GeometricFeature</Source><SourceDirection>+Z</SourceDirection><FeatureName>planar surface 32</FeatureName></PrimaryAxis><SecondaryAxis><DefinedDirection>+Y</DefinedDirection><Source>GeometricFeature</Source><SourceDirection>+X</SourceDirection><FeatureName>planar surface 33</FeatureName></SecondaryAxis></Value></Frame></Frames>
  MATLAB Function : MATLAB Function  TreatAsAtomicUnit=on
  PS-Simulink Converter : nesl_utility/PS-Simulink Converter  PhysicalDomain=network_engine_domain  SubClassName=ps_output  LeftPortType=input  RightPortType=output  PseudoPeriodic=off  Frequencies=[]  VectorFormat=inherit  Unit=inherit  AffineConversion=off
  PS-Simulink Converter1 : nesl_utility/PS-Simulink Converter  PhysicalDomain=network_engine_domain  SubClassName=ps_output  LeftPortType=input  RightPortType=output  PseudoPeriodic=off  Frequencies=[]  VectorFormat=inherit  Unit=inherit  AffineConversion=off
  Rigid Transform : sm_lib/Frames and Transforms/Rigid Transform  RotationMethod=RotationMatrix  FollAlignAxisA=+X  BaseAlignAxisA=+Y  FollAlignAxisB=+Y  BaseAlignAxisB=+Z  RotationStandardAxis=+Z  RotationAngle=0  RotationAngleUnits=deg  RotationArbitraryAxis=[0 0 1]  RotationSequenceAxes=FollowerAxes  RotationSequence=XYX  RotationSequenceAngles=[0 0 0]  RotationSequenceAnglesUnits=deg  RotationMatrix=rotLaserGate  Quaternion=[1 0 0 0]  TranslationMethod=Cartesian  TranslationCartesianOffset=posLaserGate  TranslationCartesianOffsetUnits=m  TranslationStandardAxis=+Z  TranslationStandardOffset=0  TranslationStandardOffsetUnits=m  TranslationROffset=0  TranslationROffsetUnits=m  TranslationThetaOffset=0  TranslationThetaOffsetUnits=deg  TranslationZOffset=0  TranslationZOffsetUnits=m
  Transform Sensor : sm_lib/Frames and Transforms/Transform Sensor  MeasurementFrame=World  RotationSequence=XYX  SenseAngle=off  SenseAxis=off  SenseQ=off  SenseR=on  SenseRotationSequence=off  SenseOmegaX=off  SenseOmegaY=off  SenseOmegaZ=off  SenseOmega=off  SenseQDot=off  SenseRDot=off  SenseRotationSequenceDot=off  SenseAlphaX=off  SenseAlphaY=off  SenseAlphaZ=off  SenseAlpha=off  SenseQDDot=off  SenseRDDot=off  SenseX=off  SenseY=off  SenseZ=off  SenseXYZ=on  SenseRad=off  SenseAzim=off  SenseDist=off  SenseInc=off  SenseXDot=off  SenseYDot=off  SenseZDot=off  SenseXYZDot=off  SenseRadDot=off  SenseAzimDot=off  SenseDistDot=off  SenseIncDot=off  SenseXDDot=off  SenseYDDot=off  SenseZDDot=off  SenseXYZDDot=off  SenseRadDDot=off  SenseAzimDDot=off  SenseDistDDot=off  SenseIncDDot=off
  F1 : PMIOPort  Side=Left
  LaserGate_F1 : PMIOPort  Port=2  Side=Right
  T_R_F1 : Outport
  wires:
  MATLAB Function/1(T) -> T_R_F1/1
  PS-Simulink Converter1/1 -> MATLAB Function/2(p)
  PS-Simulink Converter/1 -> MATLAB Function/1(R)
  connections:
  F1/RConn1 -- Rigid Transform/LConn1
  Rigid Transform/RConn1 -- File Solid/RConn1 -- Transform Sensor/LConn1
  Transform Sensor/RConn1 -- LaserGate_F1/RConn1 -- File Solid/LConn1
  PS-Simulink Converter/LConn1 -- Transform Sensor/RConn2
  Transform Sensor/RConn3 -- PS-Simulink Converter1/LConn1

== system macroRobot_simulator/Simulation/completeKukaRobot/Table ==
  ReferenceFrame : sm_lib/Frames and Transforms/Reference Frame
  Solid1 : sm_lib/Body Elements/Cylindrical Solid  CylinderRadius=0.25  CylinderRadiusUnits=m  CylinderLength=0.7  CylinderLengthUnits=m  ExportEntireGeometry=off  InertiaType=PointMass  BasedOnType=Density  Density=1000  DensityUnits=kg/m^3  Mass=0.001  MassUnits=kg  CenterOfMass=smiData.Solid(1).CoM  CenterOfMassUnits=mm  MomentsOfInertia=smiData.Solid(1).MoI  MomentsOfInertiaUnits=kg*mm^2  ProductsOfInertia=smiData.Solid(1).PoI  ProductsOfInertiaUnits=kg*mm^2  GraphicType=FromGeometry  MarkerShape=Sphere  MarkerSize=10  GraphicVisPropType=SimpleVisualProperties  GraphicDiffuseColor=[0.6 0.6 0.6]  GraphicOpacity=smiData.Solid(1).opacity  GraphicSpecularColor=[0.5 0.5 0.5 1.0]  GraphicAmbientColor=[0.15 0.15 0.15 1.0]  GraphicEmissiveColor=[0.0 0.0 0.0 1.0]  GraphicShininess=75  DoExposeReferenceFrame=off  SerializedFrames=<Frames><Frame><Id>Frame3</Id><Value><Name>F3</Name><Origin><Source>GeometricFeature</Source><FeatureName>top surface</FeatureName></Origin><PrimaryAxis><DefinedDirection>+Z</DefinedDirection><Source>ReferenceFrame</Source><SourceDirection>+Z</SourceDirection><FeatureName></FeatureName></PrimaryAxis><SecondaryAxis><DefinedDirection>+X</DefinedDirection><Source>ReferenceFrame</Source><SourceDirection>+X</SourceDirection><FeatureName></FeatureName></SecondaryAxis></Value></Frame></Frames>
  F1 : PMIOPort  Side=Left
  connections:
  ReferenceFrame/RConn1 -- Solid1/LConn1 -- F1/RConn1

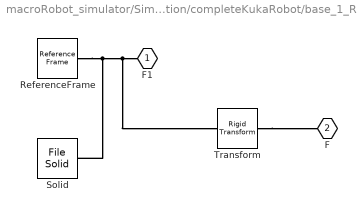
== system macroRobot_simulator/Simulation/completeKukaRobot/base_1_RIGID ==
  ReferenceFrame : sm_lib/Frames and Transforms/Reference Frame
  Solid : sm_lib/Body Elements/File Solid  ExtGeomFileName=base_Default_sldprt.STEP  UnitType=FromFile  ExtGeomFileUnits=m  StepReaderType=HEX  ExportConvexHullGeometry=off  InertiaType=Custom  BasedOnType=DensityFromFile  Density=1000  DensityUnits=kg/m^3  Mass=smiData.Solid(6).mass  MassUnits=kg  CenterOfMass=smiData.Solid(6).CoM  CenterOfMassUnits=mm  MomentsOfInertia=smiData.Solid(6).MoI  MomentsOfInertiaUnits=kg*mm^2  ProductsOfInertia=smiData.Solid(6).PoI  ProductsOfInertiaUnits=kg*mm^2  GraphicType=FromGeometry  MarkerShape=Sphere  MarkerSize=10  GraphicVisPropType=SimpleVisualProperties  GraphicDiffuseColor=smiData.Solid(6).color  GraphicOpacity=smiData.Solid(6).opacity  GraphicSpecularColor=[0.5 0.5 0.5 1.0]  GraphicAmbientColor=[0.15 0.15 0.15 1.0]  GraphicEmissiveColor=[0.0 0.0 0.0 1.0]  GraphicShininess=75  DoExposeReferenceFrame=on  SerializedFrames=<Frames/>
  Transform : sm_lib/Frames and Transforms/Rigid Transform  RotationMethod=ArbitraryAxis  FollAlignAxisA=+X  BaseAlignAxisA=+Y  FollAlignAxisB=+Y  BaseAlignAxisB=+Z  RotationStandardAxis=+Z  RotationAngle=smiData.RigidTransform(3).angle  RotationAngleUnits=rad  RotationArbitraryAxis=smiData.RigidTransform(3).axis  RotationSequenceAxes=FollowerAxes  RotationSequence=XYX  RotationSequenceAngles=[0 0 0]  RotationSequenceAnglesUnits=deg  RotationMatrix=[1 0 0; 0 1 0; 0 0 1]  Quaternion=[1 0 0 0]  TranslationMethod=Cartesian  TranslationCartesianOffset=smiData.RigidTransform(3).translation  TranslationCartesianOffsetUnits=mm  TranslationStandardAxis=+Z  TranslationStandardOffset=0  TranslationStandardOffsetUnits=m  TranslationROffset=0  TranslationROffsetUnits=m  TranslationThetaOffset=0  TranslationThetaOffsetUnits=deg  TranslationZOffset=0  TranslationZOffsetUnits=m
  F1 : PMIOPort  Side=Left
  F : PMIOPort  Port=2  Side=Right
  connections:
  ReferenceFrame/RConn1 -- Transform/LConn1 -- F1/RConn1 -- Solid/RConn1
  Transform/RConn1 -- F/RConn1

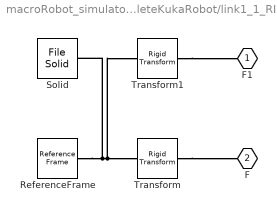
== system macroRobot_simulator/Simulation/completeKukaRobot/link1_1_RIGID ==
  ReferenceFrame : sm_lib/Frames and Transforms/Reference Frame
  Solid : sm_lib/Body Elements/File Solid  ExtGeomFileName=link1_Default_sldprt.STEP  UnitType=FromFile  ExtGeomFileUnits=m  StepReaderType=HEX  ExportConvexHullGeometry=off  InertiaType=Custom  BasedOnType=DensityFromFile  Density=1000  DensityUnits=kg/m^3  Mass=smiData.Solid(2).mass  MassUnits=kg  CenterOfMass=smiData.Solid(2).CoM  CenterOfMassUnits=mm  MomentsOfInertia=smiData.Solid(2).MoI  MomentsOfInertiaUnits=kg*mm^2  ProductsOfInertia=smiData.Solid(2).PoI  ProductsOfInertiaUnits=kg*mm^2  GraphicType=FromGeometry  MarkerShape=Sphere  MarkerSize=10  GraphicVisPropType=SimpleVisualProperties  GraphicDiffuseColor=smiData.Solid(2).color  GraphicOpacity=smiData.Solid(2).opacity  GraphicSpecularColor=[0.5 0.5 0.5 1.0]  GraphicAmbientColor=[0.15 0.15 0.15 1.0]  GraphicEmissiveColor=[0.0 0.0 0.0 1.0]  GraphicShininess=75  DoExposeReferenceFrame=on  SerializedFrames=<Frames/>
  Transform : sm_lib/Frames and Transforms/Rigid Transform  RotationMethod=ArbitraryAxis  FollAlignAxisA=+X  BaseAlignAxisA=+Y  FollAlignAxisB=+Y  BaseAlignAxisB=+Z  RotationStandardAxis=+Z  RotationAngle=smiData.RigidTransform(1).angle  RotationAngleUnits=rad  RotationArbitraryAxis=smiData.RigidTransform(1).axis  RotationSequenceAxes=FollowerAxes  RotationSequence=XYX  RotationSequenceAngles=[0 0 0]  RotationSequenceAnglesUnits=deg  RotationMatrix=[1 0 0; 0 1 0; 0 0 1]  Quaternion=[1 0 0 0]  TranslationMethod=Cartesian  TranslationCartesianOffset=smiData.RigidTransform(1).translation  TranslationCartesianOffsetUnits=mm  TranslationStandardAxis=+Z  TranslationStandardOffset=0  TranslationStandardOffsetUnits=m  TranslationROffset=0  TranslationROffsetUnits=m  TranslationThetaOffset=0  TranslationThetaOffsetUnits=deg  TranslationZOffset=0  TranslationZOffsetUnits=m
  Transform1 : sm_lib/Frames and Transforms/Rigid Transform  RotationMethod=ArbitraryAxis  FollAlignAxisA=+X  BaseAlignAxisA=+Y  FollAlignAxisB=+Y  BaseAlignAxisB=+Z  RotationStandardAxis=+Z  RotationAngle=smiData.RigidTransform(4).angle  RotationAngleUnits=rad  RotationArbitraryAxis=smiData.RigidTransform(4).axis  RotationSequenceAxes=FollowerAxes  RotationSequence=XYX  RotationSequenceAngles=[0 0 0]  RotationSequenceAnglesUnits=deg  RotationMatrix=[1 0 0; 0 1 0; 0 0 1]  Quaternion=[1 0 0 0]  TranslationMethod=Cartesian  TranslationCartesianOffset=smiData.RigidTransform(4).translation  TranslationCartesianOffsetUnits=mm  TranslationStandardAxis=+Z  TranslationStandardOffset=0  TranslationStandardOffsetUnits=m  TranslationROffset=0  TranslationROffsetUnits=m  TranslationThetaOffset=0  TranslationThetaOffsetUnits=deg  TranslationZOffset=0  TranslationZOffsetUnits=m
  F1 : PMIOPort  Side=Left
  F : PMIOPort  Port=2  Side=Right
  connections:
  ReferenceFrame/RConn1 -- Transform/LConn1 -- Transform1/LConn1 -- Solid/RConn1
  Transform/RConn1 -- F/RConn1
  Transform1/RConn1 -- F1/RConn1

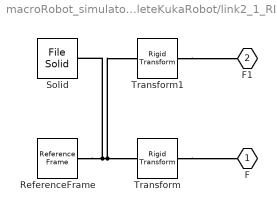
== system macroRobot_simulator/Simulation/completeKukaRobot/link2_1_RIGID ==
  ReferenceFrame : sm_lib/Frames and Transforms/Reference Frame
  Solid : sm_lib/Body Elements/File Solid  ExtGeomFileName=link2_Default_sldprt.STEP  UnitType=FromFile  ExtGeomFileUnits=m  StepReaderType=HEX  ExportConvexHullGeometry=off  InertiaType=Custom  BasedOnType=DensityFromFile  Density=1000  DensityUnits=kg/m^3  Mass=smiData.Solid(3).mass  MassUnits=kg  CenterOfMass=smiData.Solid(3).CoM  CenterOfMassUnits=mm  MomentsOfInertia=smiData.Solid(3).MoI  MomentsOfInertiaUnits=kg*mm^2  ProductsOfInertia=smiData.Solid(3).PoI  ProductsOfInertiaUnits=kg*mm^2  GraphicType=FromGeometry  MarkerShape=Sphere  MarkerSize=10  GraphicVisPropType=SimpleVisualProperties  GraphicDiffuseColor=smiData.Solid(3).color  GraphicOpacity=smiData.Solid(3).opacity  GraphicSpecularColor=[0.5 0.5 0.5 1.0]  GraphicAmbientColor=[0.15 0.15 0.15 1.0]  GraphicEmissiveColor=[0.0 0.0 0.0 1.0]  GraphicShininess=75  DoExposeReferenceFrame=on  SerializedFrames=<Frames/>
  Transform : sm_lib/Frames and Transforms/Rigid Transform  RotationMethod=ArbitraryAxis  FollAlignAxisA=+X  BaseAlignAxisA=+Y  FollAlignAxisB=+Y  BaseAlignAxisB=+Z  RotationStandardAxis=+Z  RotationAngle=smiData.RigidTransform(2).angle  RotationAngleUnits=rad  RotationArbitraryAxis=smiData.RigidTransform(2).axis  RotationSequenceAxes=FollowerAxes  RotationSequence=XYX  RotationSequenceAngles=[0 0 0]  RotationSequenceAnglesUnits=deg  RotationMatrix=[1 0 0; 0 1 0; 0 0 1]  Quaternion=[1 0 0 0]  TranslationMethod=Cartesian  TranslationCartesianOffset=smiData.RigidTransform(2).translation  TranslationCartesianOffsetUnits=mm  TranslationStandardAxis=+Z  TranslationStandardOffset=0  TranslationStandardOffsetUnits=m  TranslationROffset=0  TranslationROffsetUnits=m  TranslationThetaOffset=0  TranslationThetaOffsetUnits=deg  TranslationZOffset=0  TranslationZOffsetUnits=m
  Transform1 : sm_lib/Frames and Transforms/Rigid Transform  RotationMethod=ArbitraryAxis  FollAlignAxisA=+X  BaseAlignAxisA=+Y  FollAlignAxisB=+Y  BaseAlignAxisB=+Z  RotationStandardAxis=+Z  RotationAngle=smiData.RigidTransform(5).angle  RotationAngleUnits=rad  RotationArbitraryAxis=smiData.RigidTransform(5).axis  RotationSequenceAxes=FollowerAxes  RotationSequence=XYX  RotationSequenceAngles=[0 0 0]  RotationSequenceAnglesUnits=deg  RotationMatrix=[1 0 0; 0 1 0; 0 0 1]  Quaternion=[1 0 0 0]  TranslationMethod=Cartesian  TranslationCartesianOffset=smiData.RigidTransform(5).translation  TranslationCartesianOffsetUnits=mm  TranslationStandardAxis=+Z  TranslationStandardOffset=0  TranslationStandardOffsetUnits=m  TranslationROffset=0  TranslationROffsetUnits=m  TranslationThetaOffset=0  TranslationThetaOffsetUnits=deg  TranslationZOffset=0  TranslationZOffsetUnits=m
  F : PMIOPort  Side=Left
  F1 : PMIOPort  Port=2  Side=Right
  connections:
  ReferenceFrame/RConn1 -- Transform/LConn1 -- Transform1/LConn1 -- Solid/RConn1
  Transform/RConn1 -- F/RConn1
  Transform1/RConn1 -- F1/RConn1

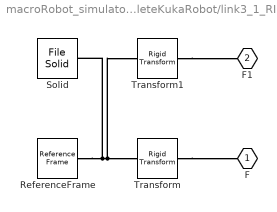
== system macroRobot_simulator/Simulation/completeKukaRobot/link3_1_RIGID ==
  ReferenceFrame : sm_lib/Frames and Transforms/Reference Frame
  Solid : sm_lib/Body Elements/File Solid  ExtGeomFileName=link3_Default_sldprt.STEP  UnitType=FromFile  ExtGeomFileUnits=m  StepReaderType=HEX  ExportConvexHullGeometry=off  InertiaType=Custom  BasedOnType=DensityFromFile  Density=1000  DensityUnits=kg/m^3  Mass=smiData.Solid(7).mass  MassUnits=kg  CenterOfMass=smiData.Solid(7).CoM  CenterOfMassUnits=mm  MomentsOfInertia=smiData.Solid(7).MoI  MomentsOfInertiaUnits=kg*mm^2  ProductsOfInertia=smiData.Solid(7).PoI  ProductsOfInertiaUnits=kg*mm^2  GraphicType=FromGeometry  MarkerShape=Sphere  MarkerSize=10  GraphicVisPropType=SimpleVisualProperties  GraphicDiffuseColor=smiData.Solid(7).color  GraphicOpacity=smiData.Solid(7).opacity  GraphicSpecularColor=[0.5 0.5 0.5 1.0]  GraphicAmbientColor=[0.15 0.15 0.15 1.0]  GraphicEmissiveColor=[0.0 0.0 0.0 1.0]  GraphicShininess=75  DoExposeReferenceFrame=on  SerializedFrames=<Frames/>
  Transform : sm_lib/Frames and Transforms/Rigid Transform  RotationMethod=ArbitraryAxis  FollAlignAxisA=+X  BaseAlignAxisA=+Y  FollAlignAxisB=+Y  BaseAlignAxisB=+Z  RotationStandardAxis=+Z  RotationAngle=smiData.RigidTransform(6).angle  RotationAngleUnits=rad  RotationArbitraryAxis=smiData.RigidTransform(6).axis  RotationSequenceAxes=FollowerAxes  RotationSequence=XYX  RotationSequenceAngles=[0 0 0]  RotationSequenceAnglesUnits=deg  RotationMatrix=[1 0 0; 0 1 0; 0 0 1]  Quaternion=[1 0 0 0]  TranslationMethod=Cartesian  TranslationCartesianOffset=smiData.RigidTransform(6).translation  TranslationCartesianOffsetUnits=mm  TranslationStandardAxis=+Z  TranslationStandardOffset=0  TranslationStandardOffsetUnits=m  TranslationROffset=0  TranslationROffsetUnits=m  TranslationThetaOffset=0  TranslationThetaOffsetUnits=deg  TranslationZOffset=0  TranslationZOffsetUnits=m
  Transform1 : sm_lib/Frames and Transforms/Rigid Transform  RotationMethod=ArbitraryAxis  FollAlignAxisA=+X  BaseAlignAxisA=+Y  FollAlignAxisB=+Y  BaseAlignAxisB=+Z  RotationStandardAxis=+Z  RotationAngle=smiData.RigidTransform(7).angle  RotationAngleUnits=rad  RotationArbitraryAxis=smiData.RigidTransform(7).axis  RotationSequenceAxes=FollowerAxes  RotationSequence=XYX  RotationSequenceAngles=[0 0 0]  RotationSequenceAnglesUnits=deg  RotationMatrix=[1 0 0; 0 1 0; 0 0 1]  Quaternion=[1 0 0 0]  TranslationMethod=Cartesian  TranslationCartesianOffset=smiData.RigidTransform(7).translation  TranslationCartesianOffsetUnits=mm  TranslationStandardAxis=+Z  TranslationStandardOffset=0  TranslationStandardOffsetUnits=m  TranslationROffset=0  TranslationROffsetUnits=m  TranslationThetaOffset=0  TranslationThetaOffsetUnits=deg  TranslationZOffset=0  TranslationZOffsetUnits=m
  F : PMIOPort  Side=Left
  F1 : PMIOPort  Port=2  Side=Right
  connections:
  ReferenceFrame/RConn1 -- Transform/LConn1 -- Transform1/LConn1 -- Solid/RConn1
  Transform/RConn1 -- F/RConn1
  Transform1/RConn1 -- F1/RConn1
